simulink model "YMBOX_Deluxe_code"  (R2024b)
settings: Solver=FixedStepDiscrete  StartTime=0.0  StopTime=20  FixedStep=Cf_CONTROL_TASK_TIME_S  RelTol=1e-3
PreLoadFcn:
  | run(fullfile(fileparts(get_param(bdroot,'FileName')), 'YMBOX_Deluxe_init.m'));
InitFcn:
  | YMBOX_InitializeModel('code',bdroot);
model workspace (MAT data in the model file):
  KfMDSP_DCBusVoltFilterCutoff_Hz = Simulink.Parameter
  KfMDSP_DCBusVoltFilterCutoff_Hz.Value = 500
  KfMDSP_DCBusVoltFilterCutoff_Hz.Complexity = 'real'
  KfMDSP_DCBusVoltFilterCutoff_Hz.Dimensions = [1 1]
  KfMDSP_DCBusVoltFilterCutoff_Hz.Description = 'DC bus voltage low-pass cutoff frequency in Hz'
  KfMDSP_DCBusVoltFilterCutoff_Hz.DataType = 'single'
  KfMDSP_DCBusVoltFilterCutoff_Hz.Min = 10
  KfMDSP_DCBusVoltFilterCutoff_Hz.Max = 1000
CloseFcn:
  | YMBOX_Deluxe_exit
settings Model: Creator=ASUS  LastModifiedBy=ASUS
settings SolverCC: AlgebraicLoopSolver=TrustRegion  AutoInsertRateTranBlk=on
settings DataIOCC: LimitDataPoints=on  SaveFormat=StructureWithTime  SignalLoggingSaveFormat=ModelDataLogs  SaveOutput=off  SaveTime=off  ReturnWorkspaceOutputs=off
settings OptimizationCC: BlockReduction=off  ConditionallyExecuteInputs=off  DefaultParameterBehavior=Inlined  DefaultUnderspecifiedDataType=single  EnhancedBackFolding=on  PassReuseOutputArgsAs=Individual arguments  ExpressionDepthLimit=2147483647  InitFltsAndDblsToZero=on  EfficientFloat2IntCast=on  EfficientMapNaN2IntZero=off  OptimizeBlockOrder=speed  DifferentSizesBufferReuse=on  OptimizationCustomize=off  EfficientTunableParamExpr=on
settings DebuggingCC: ConsistencyChecking=warning  ArrayBoundsChecking=error  SignalInfNanChecking=error  SignalRangeChecking=error  SaveWithParameterizedLinksMsg=none  CheckSSInitialOutputMsg=off  UnderspecifiedInitializationDetection=Classic  MergeDetectMultiDrivingBlocksExec=none  TimeAdjustmentMsg=warning  MaxConsecutiveZCsMsg=warning  SolverPrmCheckMsg=warning  InheritedTsInSrcMsg=none  CheckMatrixSingularityMsg=error  ParameterOverflowMsg=warning  ParameterUnderflowMsg=error  ParameterPrecisionLossMsg=none  ParameterTunabilityLossMsg=error  FixptConstUnderflowMsg=warning  FixptConstOverflowMsg=warning  FixptConstPrecisionLossMsg=warning  VectorMatrixConversionMsg=warning  FcnCallInpInsideContextMsg=warning  UnconnectedInputMsg=warning  UnconnectedOutputMsg=warning  UnconnectedLineMsg=warning  UniqueDataStoreMsg=warning  AllowSymbolicDim=off  StateNameClashWarn=warning  SFUnexpectedBacktrackingDiag=warning  SFNoUnconditionalDefaultTransitionDiag=warning  SFExecutionAtInitializationDiag=none  ArithmeticOperatorsInVariantConditions=warning
settings HardwareCC: ProdBitPerChar=16  ProdBitPerInt=16  ProdBitPerPointer=32  ProdBitPerSizeT=32  ProdBitPerPtrDiffT=32  ProdLargestAtomicInteger=Integer  ProdLargestAtomicFloat=None  ProdWordSize=16  ProdHWDeviceType=Texas Instruments->C2000  TargetIntDivRoundTo=Zero  TargetEndianess=LittleEndian  TargetHWDeviceType=Infineon->TriCore  ProdEqTarget=off
settings ModelReferenceCC: EnableRefExpFcnMdlSchedulingChecks=on  PropagateSignalLabelsOutOfModel=off
settings SFSimCC: SimUseLocalCustomCode=off  MATLABDynamicMemAlloc=off  CustomCodeUndefinedFunction=UseInterfaceOnly
settings SFSimCC: SimCustomSourceCode=|
  | void Pwm_SetOutputToIdle_Now(void){};
  | void InverterDisable(void){};
  | void Pwm_Write(void){};
  | void InverterEnable(void){};
  | void vPwm_MDCC_UdUqCalc1_PI_Self_initialize(void){};
  | void SpeedLoopMode_initialize(void){};
settings SFSimCC: SimCustomHeaderCode=|
  | void Pwm_SetOutputToIdle_Now(void);
  | void InverterDisable(void);
  | void Pwm_Write(void);
  | void InverterEnable(void);
  | void vPwm_MDCC_UdUqCalc1_PI_Self_initialize(void);
  | void SpeedLoopMode_initialize(void);
settings RTWCC: Description=Embedded Coder  SystemTargetFile=ert.tlc  TLCOptions=-p0  GenCodeOnly=on  TemplateMakefile=ert_default_tmf  GenerateReport=on  RTWUseLocalCustomCode=off  CustomHeaderCode=extern void InverterDisable(void);  IncludeHyperlinkInReport=on  LaunchReport=on  GPUComputeCapability=3.5
settings CodeAppCC: GenerateComments=off  IgnoreCustomStorageClasses=off  MaxIdLength=100  CustomSymbolStrGlobalVar=rt$N$M  CustomSymbolStrType=$N$M  CustomSymbolStrFcn=$N$M$F  CustomSymbolStrMacro=$N$M  CustomCommentsFcn=comments_mptfun.m  DefineNamingRule=UpperCase  SimulinkBlockComments=off  InternalIdentifier=Classic
settings ERTTargetCC: TargetLangStandard=C99 (ISO)  CodeReplacementLibrary=YMBOX single math  ERTCustomFileTemplate=example_file_process.tlc
settings ConfigComp: CovMetricSettings=dw  CovSaveCumulativeToWorkspaceVar=on  CovSaveSingleToWorkspaceVar=on  CovExternalEMLEnable=off

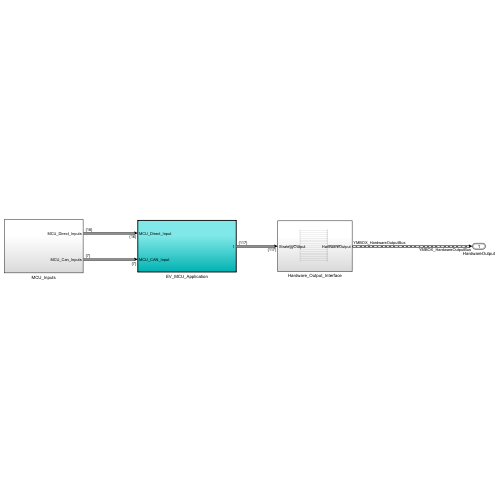
[thumbnail: Simulink's stored preview of the top-level diagram]
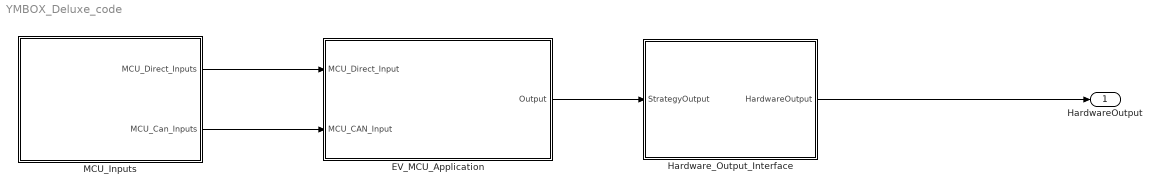
== system YMBOX_Deluxe_code ==
  EV_MCU_Application : Subsystem  TreatAsAtomicUnit=on
      settings: RTWSystemCode=Nonreusable function  RTWFcnNameOpts=Use subsystem name  RTWFileNameOpts=Use subsystem name
  Hardware_Output_Interface : Subsystem
  MCU_Inputs : Subsystem
      settings: RTWSystemCode=Nonreusable function  RTWFcnNameOpts=Use subsystem name  RTWFileNameOpts=Use subsystem name
  HardwareOutput : Outport  OutDataTypeStr=Bus: YMBOX_HardwareOutputBus
  wires:
  MCU_Inputs/1(MCU_Direct_Inputs) -> EV_MCU_Application/1(MCU_Direct_Input)
  MCU_Inputs/2(MCU_Can_Inputs) -> EV_MCU_Application/2(MCU_CAN_Input)
  EV_MCU_Application/1(Output) -> Hardware_Output_Interface/1(StrategyOutput)
  Hardware_Output_Interface/1(HardwareOutput) -> HardwareOutput/1

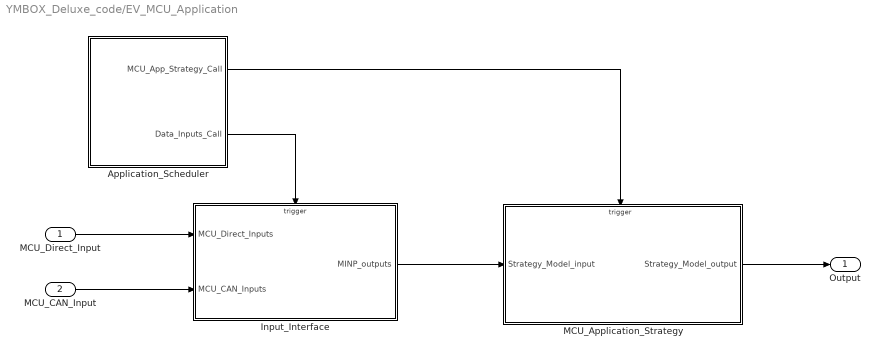
== system YMBOX_Deluxe_code/EV_MCU_Application ==
  MCU_Direct_Input : Inport
  MCU_CAN_Input : Inport  Port=2
  Application_Scheduler : Subsystem
  Input_Interface : Subsystem
      settings: RTWSystemCode=Nonreusable function  RTWFcnNameOpts=Use subsystem name  RTWFileNameOpts=Use subsystem name
  MCU_Application_Strategy : Subsystem
      settings: RTWSystemCode=Nonreusable function  RTWFcnNameOpts=Use subsystem name  RTWFileNameOpts=Use subsystem name
  Output : Outport
  wires:
  MCU_Direct_Input/1 -> Input_Interface/1(MCU_Direct_Inputs)
  MCU_CAN_Input/1 -> Input_Interface/2(MCU_CAN_Inputs)
  Input_Interface/1(MINP_outputs) -> MCU_Application_Strategy/1(Strategy_Model_input)
  MCU_Application_Strategy/1(Strategy_Model_output) -> Output/1
  Application_Scheduler/1(MCU_App_Strategy_Call) -> MCU_Application_Strategy/Trigger
  Application_Scheduler/2(Data_Inputs_Call) -> Input_Interface/Trigger

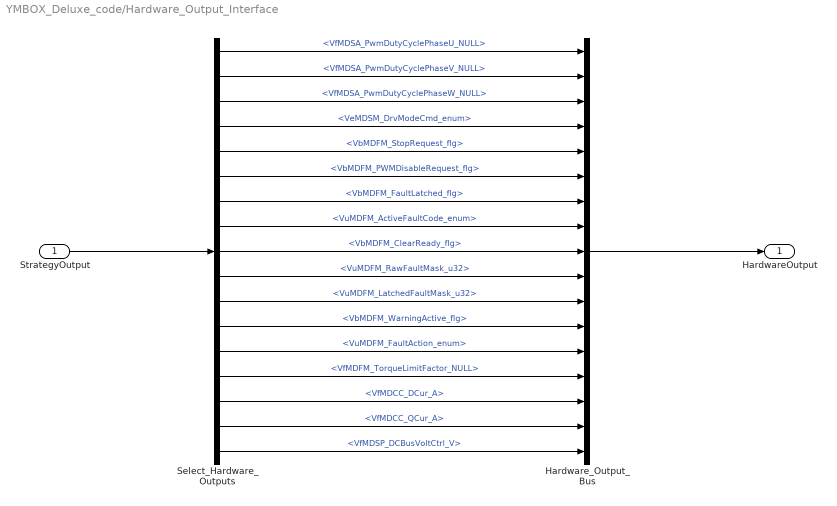
== system YMBOX_Deluxe_code/Hardware_Output_Interface ==
  StrategyOutput : Inport
  Hardware_Output_Bus : BusCreator  Inputs=17  OutDataTypeStr=Bus: YMBOX_HardwareOutputBus  NonVirtualBus=on
      settings: InheritFromInputs=off
  Select_Hardware_Outputs : BusSelector  OutputSignals=MDSA.VfMDSA_PwmDutyCyclePhaseU_NULL,MDSA.VfMDSA_PwmDutyCyclePhaseV_NULL,MDSA.VfMDSA_PwmDutyCyclePhaseW_NULL,MDSM.VeMDSM_DrvModeCmd_enum,MDFM.VbMDFM_StopRequest_flg,MDFM.VbMDFM_PWMDisableRequest_flg,MDFM.VbMDFM_FaultLatched_flg,MDFM.VuMDFM_ActiveFaultCode_enum,MDFM.VbMDFM_ClearReady_flg,MDFM.VuMDFM_RawFaultMask_u32,MDFM.VuMDFM_LatchedFaultMask_u32,MDFM.VbMDFM_WarningActive_flg,MDFM.VuMDFM_FaultAction_enum,MDFM.VfMDFM_TorqueLimitFactor_NULL,MDCC.VfMDCC_DCur_A,MDCC.VfMDCC_QCur_A,MDSP.VfMDSP_DCBusVoltCtrl_V
  HardwareOutput : Outport
  wires:
  Hardware_Output_Bus/1 -> HardwareOutput/1
  Select_Hardware_Outputs/17 -> Hardware_Output_Bus/17  "<VfMDSP_DCBusVoltCtrl_V>"
  Select_Hardware_Outputs/16 -> Hardware_Output_Bus/16  "<VfMDCC_QCur_A>"
  Select_Hardware_Outputs/15 -> Hardware_Output_Bus/15  "<VfMDCC_DCur_A>"
  Select_Hardware_Outputs/14 -> Hardware_Output_Bus/14  "<VfMDFM_TorqueLimitFactor_NULL>"
  Select_Hardware_Outputs/13 -> Hardware_Output_Bus/13  "<VuMDFM_FaultAction_enum>"
  Select_Hardware_Outputs/12 -> Hardware_Output_Bus/12  "<VbMDFM_WarningActive_flg>"
  Select_Hardware_Outputs/11 -> Hardware_Output_Bus/11  "<VuMDFM_LatchedFaultMask_u32>"
  Select_Hardware_Outputs/10 -> Hardware_Output_Bus/10  "<VuMDFM_RawFaultMask_u32>"
  Select_Hardware_Outputs/9 -> Hardware_Output_Bus/9  "<VbMDFM_ClearReady_flg>"
  Select_Hardware_Outputs/8 -> Hardware_Output_Bus/8  "<VuMDFM_ActiveFaultCode_enum>"
  Select_Hardware_Outputs/7 -> Hardware_Output_Bus/7  "<VbMDFM_FaultLatched_flg>"
  Select_Hardware_Outputs/6 -> Hardware_Output_Bus/6  "<VbMDFM_PWMDisableRequest_flg>"
  Select_Hardware_Outputs/5 -> Hardware_Output_Bus/5  "<VbMDFM_StopRequest_flg>"
  Select_Hardware_Outputs/4 -> Hardware_Output_Bus/4  "<VeMDSM_DrvModeCmd_enum>"
  Select_Hardware_Outputs/3 -> Hardware_Output_Bus/3  "<VfMDSA_PwmDutyCyclePhaseW_NULL>"
  Select_Hardware_Outputs/2 -> Hardware_Output_Bus/2  "<VfMDSA_PwmDutyCyclePhaseV_NULL>"
  Select_Hardware_Outputs/1 -> Hardware_Output_Bus/1  "<VfMDSA_PwmDutyCyclePhaseU_NULL>"
  StrategyOutput/1 -> Select_Hardware_Outputs/1

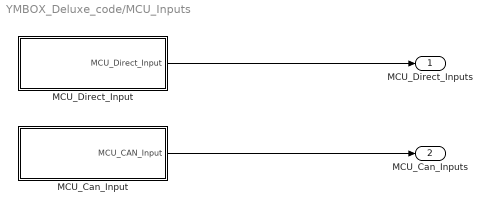
== system YMBOX_Deluxe_code/MCU_Inputs ==
  MCU_Can_Input : Subsystem  TreatAsAtomicUnit=on
      settings: RTWSystemCode=Nonreusable function  RTWFcnNameOpts=Use subsystem name
  MCU_Direct_Input : Subsystem  TreatAsAtomicUnit=on
      settings: RTWSystemCode=Nonreusable function  RTWFcnNameOpts=Use subsystem name
  MCU_Direct_Inputs : Outport
  MCU_Can_Inputs : Outport  Port=2
  wires:
  MCU_Direct_Input/1(MCU_Direct_Input) -> MCU_Direct_Inputs/1
  MCU_Can_Input/1(MCU_CAN_Input) -> MCU_Can_Inputs/1

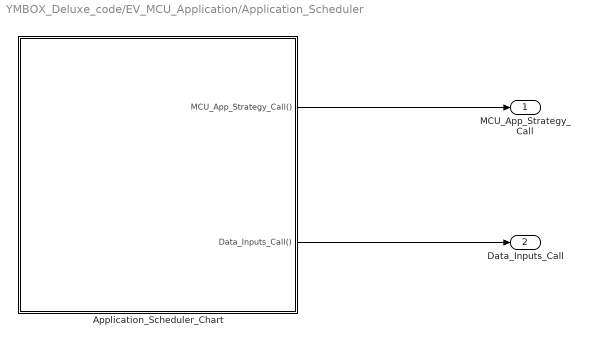
== system YMBOX_Deluxe_code/EV_MCU_Application/Application_Scheduler ==
  Application_Scheduler_Chart : Stateflow chart  TreatAsAtomicUnit=on
      settings: CopyFcn=set_param(gcb,'linkstatus','None');
  MCU_App_Strategy_Call : Outport
  Data_Inputs_Call : Outport  Port=2
  wires:
  Application_Scheduler_Chart/1(MCU_App_Strategy_Call()) -> MCU_App_Strategy_Call/1
  Application_Scheduler_Chart/2(Data_Inputs_Call()) -> Data_Inputs_Call/1

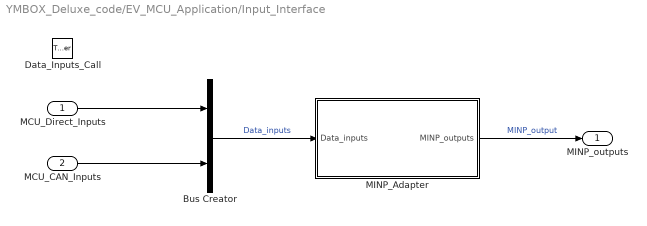
== system YMBOX_Deluxe_code/EV_MCU_Application/Input_Interface ==
  MCU_Direct_Inputs : Inport
  MCU_CAN_Inputs : Inport  Port=2
  Data_Inputs_Call : TriggerPort  TriggerType=function-call  VariantControl=(inherit)
  Bus Creator : BusCreator  Inputs=2
  MINP_Adapter : Subsystem
      settings: RTWSystemCode=Nonreusable function  RTWFcnNameOpts=Use subsystem name
  MINP_outputs : Outport  OutDataTypeStr=Bus: MINP_output
  wires:
  Bus Creator/1 -> MINP_Adapter/1(Data_inputs)  "Data_inputs"
  MCU_CAN_Inputs/1 -> Bus Creator/2
  MCU_Direct_Inputs/1 -> Bus Creator/1
  MINP_Adapter/1(MINP_outputs) -> MINP_outputs/1  "MINP_output"

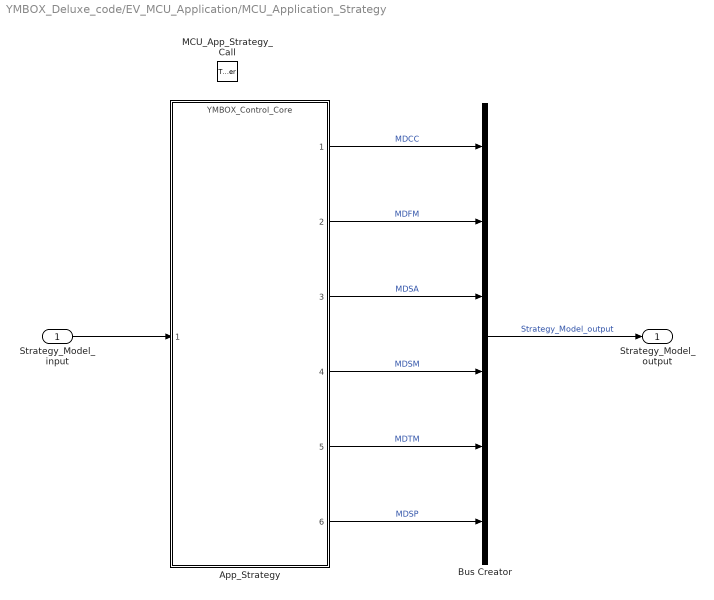
== system YMBOX_Deluxe_code/EV_MCU_Application/MCU_Application_Strategy ==
  Strategy_Model_input : Inport
  MCU_App_Strategy_Call : TriggerPort  TriggerType=function-call  VariantControl=(inherit)
  App_Strategy : ModelReference  ModelNameDialog=YMBOX_Control_Core  SimulationMode=Normal  ModelReferenceVersion=19.1094
  Bus Creator : BusCreator  Inputs=6
  Strategy_Model_output : Outport
  wires:
  Strategy_Model_input/1 -> App_Strategy/1
  Bus Creator/1 -> Strategy_Model_output/1  "Strategy_Model_output"
  App_Strategy/1 -> Bus Creator/1  "MDCC"
  App_Strategy/2 -> Bus Creator/2  "MDFM"
  App_Strategy/3 -> Bus Creator/3  "MDSA"
  App_Strategy/4 -> Bus Creator/4  "MDSM"
  App_Strategy/5 -> Bus Creator/5  "MDTM"
  App_Strategy/6 -> Bus Creator/6  "MDSP"

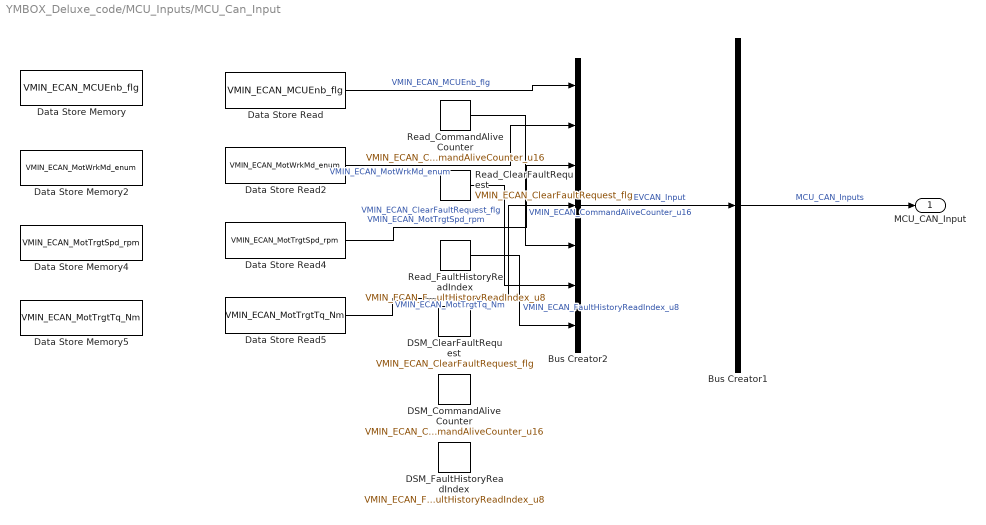
== system YMBOX_Deluxe_code/MCU_Inputs/MCU_Can_Input ==
  Bus Creator1 : BusCreator  Inputs=1
  Bus Creator2 : BusCreator  Inputs=7
  DSM_ClearFaultRequest : DataStoreMemory  DataStoreName=VMIN_ECAN_ClearFaultRequest_flg  ShowAdditionalParam=off  OutDataTypeStr=boolean  StateMustResolveToSignalObject=on
  DSM_CommandAliveCounter : DataStoreMemory  DataStoreName=VMIN_ECAN_CommandAliveCounter_u16  ShowAdditionalParam=off  OutDataTypeStr=uint16  StateMustResolveToSignalObject=on
  DSM_FaultHistoryReadIndex : DataStoreMemory  DataStoreName=VMIN_ECAN_FaultHistoryReadIndex_u8  ShowAdditionalParam=off  OutDataTypeStr=uint8  StateMustResolveToSignalObject=on
  Data Store Memory : DataStoreMemory  DataStoreName=VMIN_ECAN_MCUEnb_flg  WriteAfterWriteMsg=warning  ShowAdditionalParam=off  OutDataTypeStr=boolean  StateMustResolveToSignalObject=on
  Data Store Memory2 : DataStoreMemory  DataStoreName=VMIN_ECAN_MotWrkMd_enum  WriteAfterWriteMsg=warning  ShowAdditionalParam=off  OutDataTypeStr=uint16  StateMustResolveToSignalObject=on
  Data Store Memory4 : DataStoreMemory  DataStoreName=VMIN_ECAN_MotTrgtSpd_rpm  WriteAfterWriteMsg=warning  ShowAdditionalParam=off  OutDataTypeStr=single  StateMustResolveToSignalObject=on
  Data Store Memory5 : DataStoreMemory  DataStoreName=VMIN_ECAN_MotTrgtTq_Nm  WriteAfterWriteMsg=warning  ShowAdditionalParam=off  OutDataTypeStr=single  StateMustResolveToSignalObject=on
  Data Store Read : DataStoreRead  DataStoreName=VMIN_ECAN_MCUEnb_flg  IndexOptions=Index vector (dialog)  Indices=1  OutputSizes=1
  Data Store Read2 : DataStoreRead  DataStoreName=VMIN_ECAN_MotWrkMd_enum  IndexOptions=Index vector (dialog)  Indices=1  OutputSizes=1
  Data Store Read4 : DataStoreRead  DataStoreName=VMIN_ECAN_MotTrgtSpd_rpm  IndexOptions=Index vector (dialog)  Indices=1  OutputSizes=1
  Data Store Read5 : DataStoreRead  DataStoreName=VMIN_ECAN_MotTrgtTq_Nm  IndexOptions=Index vector (dialog)  Indices=1  OutputSizes=1
  Read_ClearFaultRequest : DataStoreRead  DataStoreName=VMIN_ECAN_ClearFaultRequest_flg  IndexOptions=Index vector (dialog)  Indices=1  OutputSizes=1
  Read_CommandAliveCounter : DataStoreRead  DataStoreName=VMIN_ECAN_CommandAliveCounter_u16  IndexOptions=Index vector (dialog)  Indices=1  OutputSizes=1
  Read_FaultHistoryReadIndex : DataStoreRead  DataStoreName=VMIN_ECAN_FaultHistoryReadIndex_u8  IndexOptions=Index vector (dialog)  Indices=1  OutputSizes=1
  MCU_CAN_Input : Outport
  wires:
  Bus Creator2/1 -> Bus Creator1/1  "EVCAN_Input"
  Bus Creator1/1 -> MCU_CAN_Input/1  "MCU_CAN_Inputs"
  Data Store Read/1 -> Bus Creator2/1  "VMIN_ECAN_MCUEnb_flg"
  Data Store Read2/1 -> Bus Creator2/2  "VMIN_ECAN_MotWrkMd_enum"
  Data Store Read4/1 -> Bus Creator2/3  "VMIN_ECAN_MotTrgtSpd_rpm"
  Data Store Read5/1 -> Bus Creator2/4  "VMIN_ECAN_MotTrgtTq_Nm"
  Read_CommandAliveCounter/1 -> Bus Creator2/5  "VMIN_ECAN_CommandAliveCounter_u16"
  Read_ClearFaultRequest/1 -> Bus Creator2/6  "VMIN_ECAN_ClearFaultRequest_flg"
  Read_FaultHistoryReadIndex/1 -> Bus Creator2/7  "VMIN_ECAN_FaultHistoryReadIndex_u8"

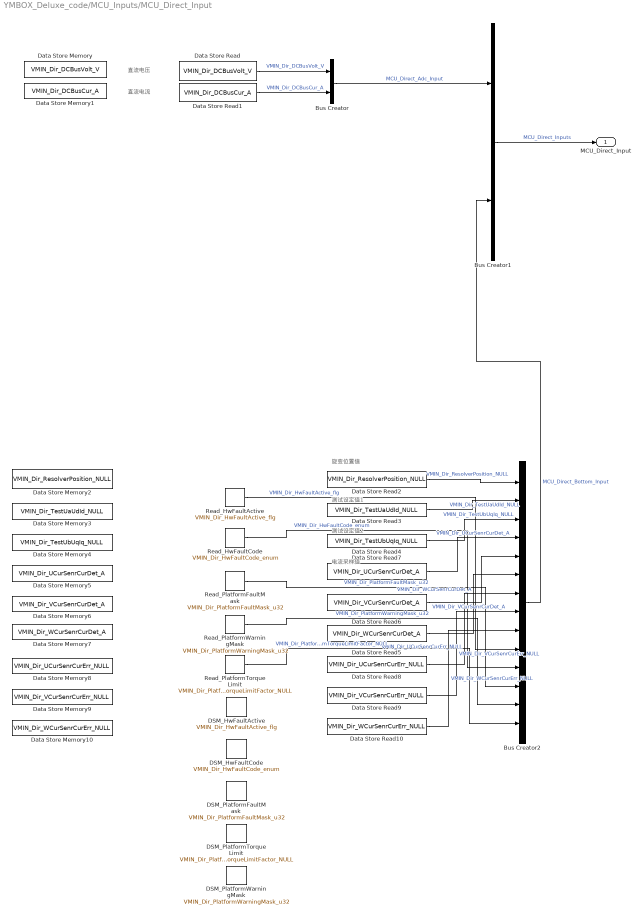
== system YMBOX_Deluxe_code/MCU_Inputs/MCU_Direct_Input ==
  note: 直流电压
  note: 直流电流
  note: 旋变位置值
  note: 测试设定值1
  note: 测试设定值2
  note: 电流采样值
  Bus Creator : BusCreator  Inputs=2
  Bus Creator1 : BusCreator  Inputs=2
  Bus Creator2 : BusCreator  Inputs=14
  DSM_HwFaultActive : DataStoreMemory  DataStoreName=VMIN_Dir_HwFaultActive_flg  ShowAdditionalParam=off  OutDataTypeStr=boolean  StateMustResolveToSignalObject=on
  DSM_HwFaultCode : DataStoreMemory  DataStoreName=VMIN_Dir_HwFaultCode_enum  ShowAdditionalParam=off  OutDataTypeStr=uint16  StateMustResolveToSignalObject=on
  DSM_PlatformFaultMask : DataStoreMemory  DataStoreName=VMIN_Dir_PlatformFaultMask_u32  ShowAdditionalParam=off  OutDataTypeStr=uint32  StateMustResolveToSignalObject=on
  DSM_PlatformTorqueLimit : DataStoreMemory  DataStoreName=VMIN_Dir_PlatformTorqueLimitFactor_NULL  InitialValue=1  ShowAdditionalParam=off  OutDataTypeStr=single  StateMustResolveToSignalObject=on
  DSM_PlatformWarningMask : DataStoreMemory  DataStoreName=VMIN_Dir_PlatformWarningMask_u32  ShowAdditionalParam=off  OutDataTypeStr=uint32  StateMustResolveToSignalObject=on
  Data Store Memory : DataStoreMemory  DataStoreName=VMIN_Dir_DCBusVolt_V  WriteAfterWriteMsg=warning  ShowAdditionalParam=off  OutDataTypeStr=single  StateMustResolveToSignalObject=on
  Data Store Memory1 : DataStoreMemory  DataStoreName=VMIN_Dir_DCBusCur_A  WriteAfterWriteMsg=warning  ShowAdditionalParam=off  OutDataTypeStr=single  StateMustResolveToSignalObject=on
  Data Store Memory10 : DataStoreMemory  DataStoreName=VMIN_Dir_WCurSenrCurErr_NULL  WriteAfterWriteMsg=warning  ShowAdditionalParam=off  OutDataTypeStr=boolean  StateMustResolveToSignalObject=on
  Data Store Memory2 : DataStoreMemory  DataStoreName=VMIN_Dir_ResolverPosition_NULL  WriteAfterWriteMsg=warning  ShowAdditionalParam=off  OutDataTypeStr=uint32  StateMustResolveToSignalObject=on
  Data Store Memory3 : DataStoreMemory  DataStoreName=VMIN_Dir_TestUaUdId_NULL  WriteAfterWriteMsg=warning  ShowAdditionalParam=off  OutDataTypeStr=single  StateMustResolveToSignalObject=on
  Data Store Memory4 : DataStoreMemory  DataStoreName=VMIN_Dir_TestUbUqIq_NULL  WriteAfterWriteMsg=warning  ShowAdditionalParam=off  OutDataTypeStr=single  StateMustResolveToSignalObject=on
  Data Store Memory5 : DataStoreMemory  DataStoreName=VMIN_Dir_UCurSenrCurDet_A  WriteAfterWriteMsg=warning  ShowAdditionalParam=off  OutDataTypeStr=single  StateMustResolveToSignalObject=on
  Data Store Memory6 : DataStoreMemory  DataStoreName=VMIN_Dir_VCurSenrCurDet_A  WriteAfterWriteMsg=warning  ShowAdditionalParam=off  OutDataTypeStr=single  StateMustResolveToSignalObject=on
  Data Store Memory7 : DataStoreMemory  DataStoreName=VMIN_Dir_WCurSenrCurDet_A  WriteAfterWriteMsg=warning  ShowAdditionalParam=off  OutDataTypeStr=single  StateMustResolveToSignalObject=on
  Data Store Memory8 : DataStoreMemory  DataStoreName=VMIN_Dir_UCurSenrCurErr_NULL  WriteAfterWriteMsg=warning  ShowAdditionalParam=off  OutDataTypeStr=boolean  StateMustResolveToSignalObject=on
  Data Store Memory9 : DataStoreMemory  DataStoreName=VMIN_Dir_VCurSenrCurErr_NULL  WriteAfterWriteMsg=warning  ShowAdditionalParam=off  OutDataTypeStr=boolean  StateMustResolveToSignalObject=on
  Data Store Read : DataStoreRead  DataStoreName=VMIN_Dir_DCBusVolt_V  IndexOptions=Index vector (dialog)  Indices=1  OutputSizes=1
  Data Store Read1 : DataStoreRead  DataStoreName=VMIN_Dir_DCBusCur_A  IndexOptions=Index vector (dialog)  Indices=1  OutputSizes=1
  Data Store Read10 : DataStoreRead  DataStoreName=VMIN_Dir_WCurSenrCurErr_NULL  IndexOptions=Index vector (dialog)  Indices=1  OutputSizes=1
  Data Store Read2 : DataStoreRead  DataStoreName=VMIN_Dir_ResolverPosition_NULL  IndexOptions=Index vector (dialog)  Indices=1  OutputSizes=1
  Data Store Read3 : DataStoreRead  DataStoreName=VMIN_Dir_TestUaUdId_NULL  IndexOptions=Index vector (dialog)  Indices=1  OutputSizes=1
  Data Store Read4 : DataStoreRead  DataStoreName=VMIN_Dir_TestUbUqIq_NULL  IndexOptions=Index vector (dialog)  Indices=1  OutputSizes=1
  Data Store Read5 : DataStoreRead  DataStoreName=VMIN_Dir_WCurSenrCurDet_A  IndexOptions=Index vector (dialog)  Indices=1  OutputSizes=1
  Data Store Read6 : DataStoreRead  DataStoreName=VMIN_Dir_VCurSenrCurDet_A  IndexOptions=Index vector (dialog)  Indices=1  OutputSizes=1
  Data Store Read7 : DataStoreRead  DataStoreName=VMIN_Dir_UCurSenrCurDet_A  IndexOptions=Index vector (dialog)  Indices=1  OutputSizes=1
  Data Store Read8 : DataStoreRead  DataStoreName=VMIN_Dir_UCurSenrCurErr_NULL  IndexOptions=Index vector (dialog)  Indices=1  OutputSizes=1
  Data Store Read9 : DataStoreRead  DataStoreName=VMIN_Dir_VCurSenrCurErr_NULL  IndexOptions=Index vector (dialog)  Indices=1  OutputSizes=1
  Read_HwFaultActive : DataStoreRead  DataStoreName=VMIN_Dir_HwFaultActive_flg  IndexOptions=Index vector (dialog)  Indices=1  OutputSizes=1
  Read_HwFaultCode : DataStoreRead  DataStoreName=VMIN_Dir_HwFaultCode_enum  IndexOptions=Index vector (dialog)  Indices=1  OutputSizes=1
  Read_PlatformFaultMask : DataStoreRead  DataStoreName=VMIN_Dir_PlatformFaultMask_u32  IndexOptions=Index vector (dialog)  Indices=1  OutputSizes=1
  Read_PlatformTorqueLimit : DataStoreRead  DataStoreName=VMIN_Dir_PlatformTorqueLimitFactor_NULL  IndexOptions=Index vector (dialog)  Indices=1  OutputSizes=1
  Read_PlatformWarningMask : DataStoreRead  DataStoreName=VMIN_Dir_PlatformWarningMask_u32  IndexOptions=Index vector (dialog)  Indices=1  OutputSizes=1
  MCU_Direct_Input : Outport
  wires:
  Data Store Read/1 -> Bus Creator/1  "VMIN_Dir_DCBusVolt_V"
  Data Store Read1/1 -> Bus Creator/2  "VMIN_Dir_DCBusCur_A"
  Bus Creator/1 -> Bus Creator1/1  "MCU_Direct_Adc_Input"
  Bus Creator1/1 -> MCU_Direct_Input/1  "MCU_Direct_Inputs"
  Data Store Read2/1 -> Bus Creator2/1  "VMIN_Dir_ResolverPosition_NULL"
  Data Store Read3/1 -> Bus Creator2/2  "VMIN_Dir_TestUaUdId_NULL"
  Data Store Read4/1 -> Bus Creator2/3  "VMIN_Dir_TestUbUqIq_NULL"
  Bus Creator2/1 -> Bus Creator1/2  "MCU_Direct_Bottom_Input"
  Data Store Read6/1 -> Bus Creator2/5  "VMIN_Dir_VCurSenrCurDet_A"
  Data Store Read7/1 -> Bus Creator2/4  "VMIN_Dir_UCurSenrCurDet_A"
  Data Store Read5/1 -> Bus Creator2/6  "VMIN_Dir_WCurSenrCurDet_A"
  Data Store Read10/1 -> Bus Creator2/9  "VMIN_Dir_WCurSenrCurErr_NULL"
  Data Store Read8/1 -> Bus Creator2/7  "VMIN_Dir_UCurSenrCurErr_NULL"
  Data Store Read9/1 -> Bus Creator2/8  "VMIN_Dir_VCurSenrCurErr_NULL"
  Read_HwFaultActive/1 -> Bus Creator2/10  "VMIN_Dir_HwFaultActive_flg"
  Read_HwFaultCode/1 -> Bus Creator2/11  "VMIN_Dir_HwFaultCode_enum"
  Read_PlatformFaultMask/1 -> Bus Creator2/12  "VMIN_Dir_PlatformFaultMask_u32"
  Read_PlatformWarningMask/1 -> Bus Creator2/13  "VMIN_Dir_PlatformWarningMask_u32"
  Read_PlatformTorqueLimit/1 -> Bus Creator2/14  "VMIN_Dir_PlatformTorqueLimitFactor_NULL"

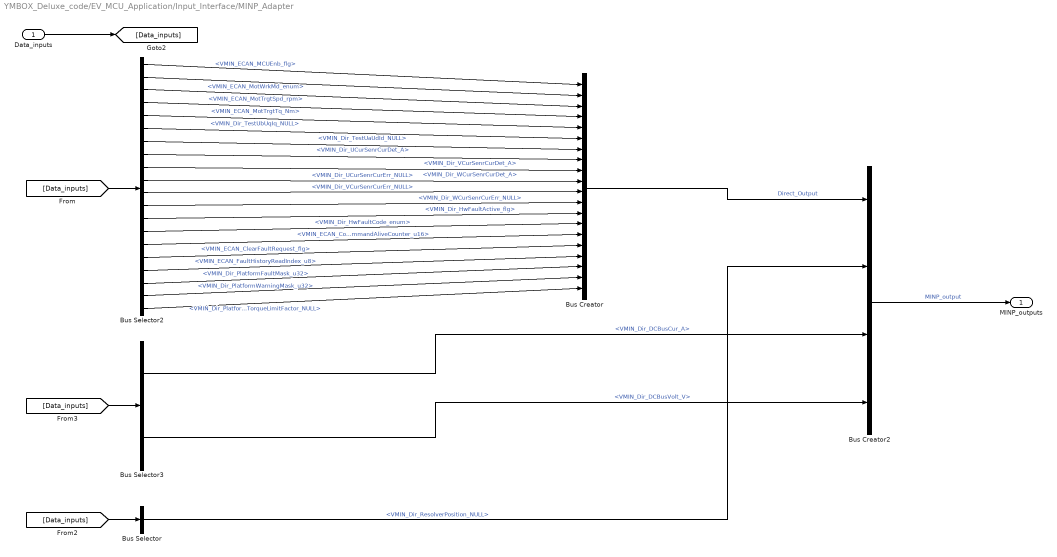
== system YMBOX_Deluxe_code/EV_MCU_Application/Input_Interface/MINP_Adapter ==
  Data_inputs : Inport
  Bus Creator : BusCreator  Inputs=20  OutDataTypeStr=Bus: Direct_Output  NonVirtualBus=on
      settings: InheritFromInputs=off
  Bus Creator2 : BusCreator  Inputs=4  OutDataTypeStr=Bus: MINP_output  NonVirtualBus=on
      settings: InheritFromInputs=off
  Bus Selector : BusSelector  OutputSignals=MCU_Direct_Inputs.MCU_Direct_Bottom_Input.VMIN_Dir_ResolverPosition_NULL
  Bus Selector2 : BusSelector  OutputSignals=MCU_CAN_Inputs.EVCAN_Input.VMIN_ECAN_MCUEnb_flg,MCU_CAN_Inputs.EVCAN_Input.VMIN_ECAN_MotWrkMd_enum,MCU_CAN_Inputs.EVCAN_Input.VMIN_ECAN_MotTrgtSpd_rpm,MCU_CAN_Inputs.EVCAN_Input.VMIN_ECAN_MotTrgtTq_Nm,MCU_Direct_Inputs.MCU_Direct_Bottom_Input.VMIN_Dir_TestUbUqIq_NULL,MCU_Direct_Inputs.MCU_Direct_Bottom_Input.VMIN_Dir_TestUaUdId_NULL,MCU_Direct_Inputs.MCU_Direct_Bottom_Input.VMIN_Dir_UCurSenrCurDet_A,MCU_Direct_Inputs.MCU_Direct_Bottom_Input.VMIN_Dir_VCurSenrCurDet_A,MCU_Direct_Inputs.MCU_Direct_Bottom_Input.VMIN_Dir_WCurSenrCurDet_A,MCU_Direct_Inputs.MCU_Direct_Bottom_Input.VMIN_Dir_UCurSenrCurErr_NULL,MCU_Direct_Inputs.MCU_Direct_Bottom_Input.VMIN_Dir_VCurSenrCurErr_NULL,MCU_Direct_Inputs.MCU_Direct_Bottom_Input.VMIN_Dir_WCurSenrCurErr_NULL,MCU_Direct_Inputs.MCU_Direct_Bottom_Input.VMIN_Dir_HwFaultActive_flg,MCU_Direct_Inputs.MCU_Direct_Bottom_Input.VMIN_Dir_HwFaultCode_enum,MCU_CAN_Inputs.EVCAN_Input.VMIN_ECAN_CommandAliveCounter_u16,MCU_CAN_Inputs.EVCAN_Input.VMIN_ECAN_ClearFaultRequest_flg,MCU_CAN_Inputs.EVCAN_Input.VMIN_ECAN_FaultHistoryReadIndex_u8,MCU_Direct_Inputs.MCU_Direct_Bottom_Input.VMIN_Dir_PlatformFaultMask_u32,MCU_Direct_Inputs.MCU_Direct_Bottom_Input.VMIN_Dir_PlatformWarningMask_u32,MCU_Direct_Inputs.MCU_Direct_Bottom_Input.VMIN_Dir_PlatformTorqueLimitFactor_NULL
  Bus Selector3 : BusSelector  OutputSignals=MCU_Direct_Inputs.MCU_Direct_Adc_Input.VMIN_Dir_DCBusCur_A,MCU_Direct_Inputs.MCU_Direct_Adc_Input.VMIN_Dir_DCBusVolt_V
  MINP_outputs : Outport  OutDataTypeStr=Bus: MINP_output
  wires:
  Data_inputs/1 -> [Data_inputs]
  [Data_inputs] -> Bus Selector2/1
  Bus Selector2/1 -> Bus Creator/1  "<VMIN_ECAN_MCUEnb_flg>"
  Bus Selector2/2 -> Bus Creator/2  "<VMIN_ECAN_MotWrkMd_enum>"
  Bus Selector2/3 -> Bus Creator/3  "<VMIN_ECAN_MotTrgtSpd_rpm>"
  Bus Selector2/5 -> Bus Creator/5  "<VMIN_Dir_TestUbUqIq_NULL>"
  Bus Selector2/6 -> Bus Creator/6  "<VMIN_Dir_TestUaUdId_NULL>"
  Bus Selector2/7 -> Bus Creator/7  "<VMIN_Dir_UCurSenrCurDet_A>"
  Bus Selector2/8 -> Bus Creator/8  "<VMIN_Dir_VCurSenrCurDet_A>"
  Bus Selector2/9 -> Bus Creator/9  "<VMIN_Dir_WCurSenrCurDet_A>"
  [Data_inputs] -> Bus Selector3/1
  Bus Selector2/4 -> Bus Creator/4  "<VMIN_ECAN_MotTrgtTq_Nm>"
  Bus Creator/1 -> Bus Creator2/1  "Direct_Output"
  Bus Creator2/1 -> MINP_outputs/1  "MINP_output"
  [Data_inputs] -> Bus Selector/1
  Bus Selector2/10 -> Bus Creator/10  "<VMIN_Dir_UCurSenrCurErr_NULL>"
  Bus Selector2/11 -> Bus Creator/11  "<VMIN_Dir_VCurSenrCurErr_NULL>"
  Bus Selector2/12 -> Bus Creator/12  "<VMIN_Dir_WCurSenrCurErr_NULL>"
  Bus Selector2/13 -> Bus Creator/13  "<VMIN_Dir_HwFaultActive_flg>"
  Bus Selector2/14 -> Bus Creator/14  "<VMIN_Dir_HwFaultCode_enum>"
  Bus Selector2/15 -> Bus Creator/15  "<VMIN_ECAN_CommandAliveCounter_u16>"
  Bus Selector2/16 -> Bus Creator/16  "<VMIN_ECAN_ClearFaultRequest_flg>"
  Bus Selector2/17 -> Bus Creator/17  "<VMIN_ECAN_FaultHistoryReadIndex_u8>"
  Bus Selector2/18 -> Bus Creator/18  "<VMIN_Dir_PlatformFaultMask_u32>"
  Bus Selector2/19 -> Bus Creator/19  "<VMIN_Dir_PlatformWarningMask_u32>"
  Bus Selector2/20 -> Bus Creator/20  "<VMIN_Dir_PlatformTorqueLimitFactor_NULL>"
  Bus Selector/1 -> Bus Creator2/2  "<VMIN_Dir_ResolverPosition_NULL>"
  Bus Selector3/1 -> Bus Creator2/3  "<VMIN_Dir_DCBusCur_A>"
  Bus Selector3/2 -> Bus Creator2/4  "<VMIN_Dir_DCBusVolt_V>"

== stateflow chart YMBOX_Deluxe_code/EV_MCU_Application/Application_Scheduler/Application_Scheduler_Chart ==
  settings: updateMethod=DISCRETE  sampleTime=Cf_CONTROL_TASK_TIME_S
  (default) -> (junction 113)
  (junction 113) -> (junction 114) : {
      |   Data_Inputs_Call;
      |   MCU_App_Strategy_Call;
      | }
  events: MCU_App_Strategy_Call output FUNCTION_CALL_EVENT; Data_Inputs_Call output FUNCTION_CALL_EVENT
